simulink model "task2"  (R2024b)
settings: Solver=VariableStepAuto  StartTime=0.0  StopTime=10.0  RelTol=1e-3
settings Model: Creator=33657  LastModifiedBy=33657

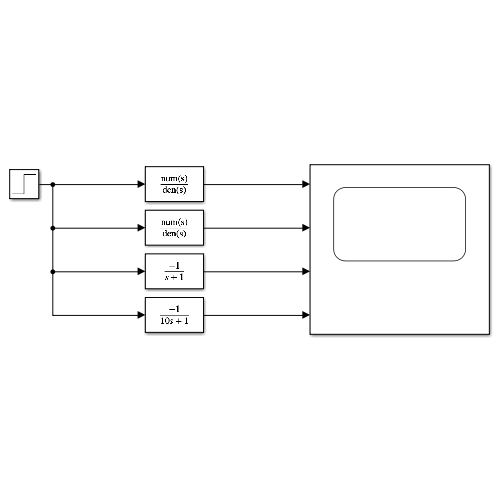
[thumbnail: Simulink's stored preview of the top-level diagram]
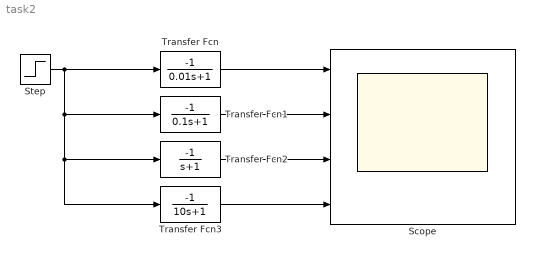
== system task2 ==
  Scope : Scope  NumInputPorts=4
  Step : Step  SampleTime=0
  Transfer Fcn : TransferFcn  Numerator=[-1]  Denominator=[0.01 1]
  Transfer Fcn1 : TransferFcn  Numerator=[-1]  Denominator=[0.1 1]
  Transfer Fcn2 : TransferFcn  Numerator=[-1]  Denominator=[1 1]
  Transfer Fcn3 : TransferFcn  Numerator=[-1]  Denominator=[10 1]
  wires:
  Step/1 -> Transfer Fcn3/1, Transfer Fcn2/1, Transfer Fcn1/1, Transfer Fcn/1
  Transfer Fcn/1 -> Scope/1
  Transfer Fcn1/1 -> Scope/2
  Transfer Fcn2/1 -> Scope/3
  Transfer Fcn3/1 -> Scope/4
